simulink model "day01_kinematics"  (R2024a)
settings: Solver=ode45  StartTime=0.0  StopTime=4  MaxStep=0.01  RelTol=1e-3
settings Model: Creator=admin  LastModifiedBy=admin

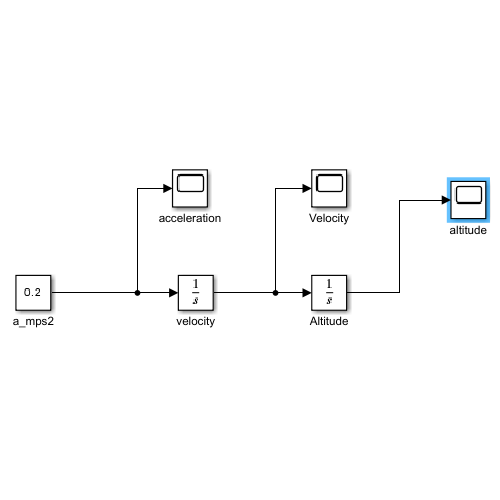
[thumbnail: Simulink's stored preview of the top-level diagram]
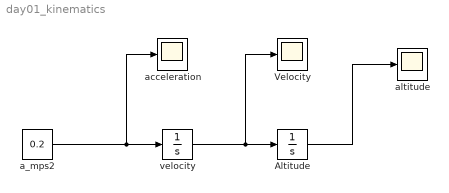
== system day01_kinematics ==
  Altitude : Integrator
  Velocity : Scope
  a_mps2 : Constant  Value=0.2
  acceleration : Scope
  altitude : Scope
  velocity : Integrator
  wires:
  a_mps2/1 -> acceleration/1, velocity/1
  velocity/1 -> Velocity/1, Altitude/1
  Altitude/1 -> altitude/1
